simulink model "HW1_7_DOB_r1_no"  (R2025a)
settings: Solver=VariableStepAuto  StartTime=0.0  StopTime=5  RelTol=1e-3
settings Model: Creator=BCC  LastModifiedBy=BCC

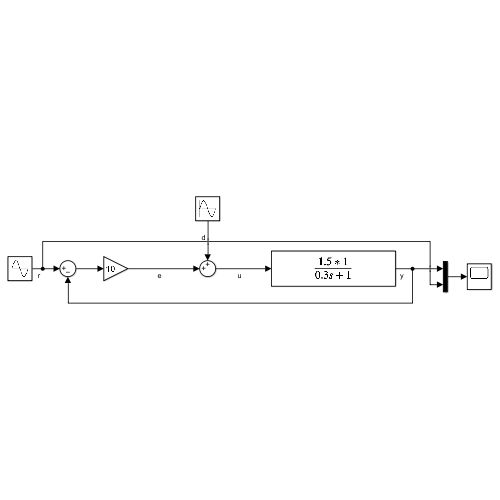
[thumbnail: Simulink's stored preview of the top-level diagram]
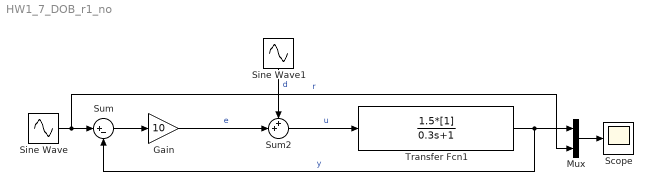
== system HW1_7_DOB_r1_no ==
  Gain : Gain  Gain=10
  Mux : Mux  Inputs=2
  Scope : Scope
      settings: ActiveDisplayYMinimum=-1.7538217253697685  ActiveDisplayYMaximum=1.751561250264799
  Sine Wave : Sin  Frequency=2*pi*2  SampleTime=0
  Sine Wave1 : Sin  Amplitude=5  Frequency=2*pi*26  SampleTime=0
  Sum : Sum  Inputs=|+-
  Sum2 : Sum  Inputs=++|  CollapseMode=Specified dimension  CollapseDim=2
  Transfer Fcn1 : TransferFcn  Numerator=1.5*[1]  Denominator=[0.3 1]
  wires:
  Sine Wave/1 -> Mux/2, Sum/1  "r"
  Sum/1 -> Gain/1
  Gain/1 -> Sum2/2  "e"
  Transfer Fcn1/1 -> Mux/1, Sum/2  "y"
  Sine Wave1/1 -> Sum2/1  "d"
  Sum2/1 -> Transfer Fcn1/1  "u"
  Mux/1 -> Scope/1
